simulink model "straperr"  (Simulink 7.9)
settings: Solver=ode23s  StartTime=0.0  StopTime=793  FixedStep=1  RelTol=1e-3
undefined symbols (not defined in the file or in its folder): D0, dcm2lat, dcm2lon, dcm2pitch, dcm2roll, dcm2yaw, getElem, plumbbobg, skew
libraries: simulink x2
settings Model: Creator=mcar  LastModifiedBy=1104070  ExtModeAutoUpdateStatusClock=off  BufferReuse=off
settings DataIOCC: ExternalInput=tu  LoadExternalInput=on  SaveFormat=StructureWithTime  SignalLoggingName=sigsOut
settings OptimizationCC: BlockReduction=off  BooleanDataType=off  OptimizeBlockIOStorage=off  BufferReuse=off  ExpressionFolding=off  LocalBlockOutputs=off
settings DebuggingCC: SaveWithParameterizedLinksMsg=none  SignalResolutionControl=TryResolveAllWithWarning  SolverPrmCheckMsg=none  MultiTaskDSMMsg=warning  MultiTaskCondExecSysMsg=none  StrictBusMsg=None
settings HardwareCC: TargetUnknown=on
settings RTWCC: IncludeERTFirstTime=on
settings GRTTargetCC: CombineOutputUpdateFcns=off  GRTInterface=on

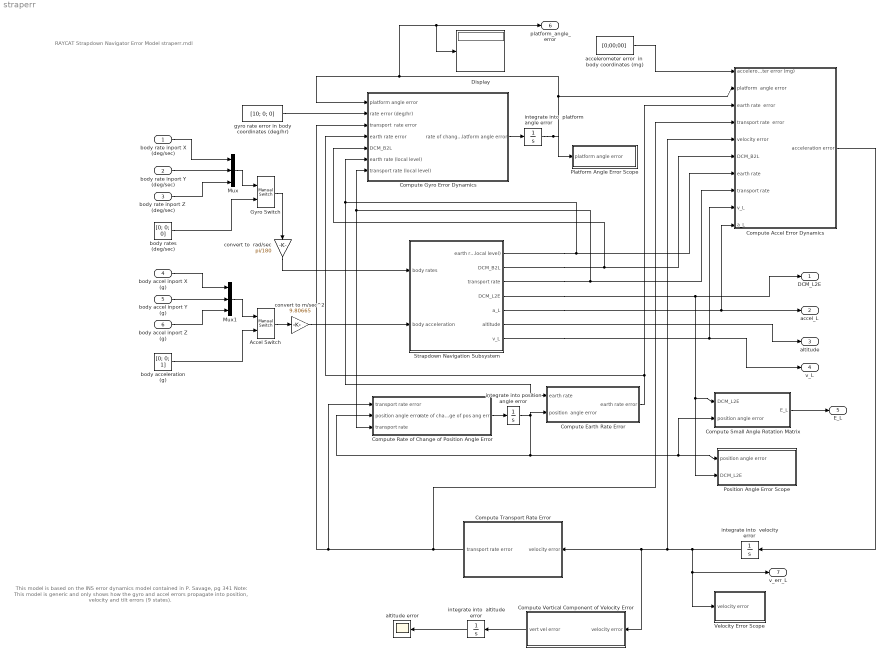
== system straperr ==
  note: RAYCAT Strapdown Navigator Error Model
      | straperr.mdl
  note: This model is based on the INS
      | error dynamics model contained in P. Savage, pg 341
      | Note:  This model is generic and only
      | shows how the gyro and accel errors propagate
      | into position, velocity and tilt errors (9 states).
  body rate inport X (deg/sec) : Inport
  body rate inport Y (deg/sec) : Inport  Port=2
  body rate inport Z  (deg/sec) : Inport  Port=3
  body accel inport X (g) : Inport  Port=4
  body accel inport Y (g) : Inport  Port=5
  body accel inport Z (g) : Inport  Port=6
  Accel Switch : simulink/Signal Routing/Manual Switch  sw=1  action=0  varsize=off
  Compute Accel Error Dynamics : Subsystem
  Compute Earth Rate Error : Subsystem
  Compute Gyro Error Dynamics : Subsystem
  Compute Rate of Change of Position Angle Error : Subsystem
  Compute Small Angle Rotation Matrix : Subsystem
  Compute Transport Rate Error : Subsystem
  Compute Vertical Component of Velocity Error : Subsystem
  Display : Display
  Gyro Switch : simulink/Signal Routing/Manual Switch  sw=1  action=0  varsize=off
  Mux : Mux  Inputs=3
  Mux1 : Mux  Inputs=3
  Platform Angle Error Scope : Subsystem
  Position Angle Error Scope : Subsystem
  Strapdown Navigation Subsystem : Subsystem  AncestorBlock=strapnavlib/Strapdown Navigation Subsystem
  Velocity Error Scope : Subsystem
  accelerometer error  in body coordinates (mg) : Constant  Value=[0;00;00]  VectorParams1D=off
  altitude error : Scope
      settings: YMin=-1  YMax=1
  body acceleration (g) : Constant  Value=[0; 0; 1]  VectorParams1D=off
  body rates (deg/sec) : Constant  Value="[0; 0;  0]"  VectorParams1D=off
  convert to  rad/sec : Gain  Gain=pi/180  SaturateOnIntegerOverflow=on  OutDataTypeStr=Inherit: Same as input  ParamDataTypeStr=Inherit: Same as input
  convert to m/sec^2 : Gain  Gain=9.80665  SaturateOnIntegerOverflow=on  OutDataTypeStr=Inherit: Same as input  ParamDataTypeStr=Inherit: Same as input
  gyro rate error in body coordinates (deg/hr) : Constant  Value=[10; 0; 0]  VectorParams1D=off
  integrate into position angle error : Integrator  InitialCondition=[0;0;0]
  integrate into  altitude error : Integrator  InitialCondition=[0;0;0]
  integrate into  platform angle error : Integrator  InitialCondition=[0;0;0]
  integrate into  velocity error : Integrator  InitialCondition=[0;0;0]
  DCM_L2E : Outport
  accel_L : Outport  Port=2
  altitude : Outport  Port=3
  v_L : Outport  Port=4
  E_L : Outport  Port=5
  platform_angle_error : Outport  Port=6
  v_err_L : Outport  Port=7
  wires:
  gyro rate error in body coordinates (deg/hr)/1 -> Compute Gyro Error Dynamics/2(rate error (deg/hr))
  Compute Gyro Error Dynamics/1(rate of change of platform angle error) -> integrate into  platform angle error/1
  integrate into  platform angle error/1 -> Platform Angle Error Scope/1(platform angle error), Compute Accel Error Dynamics/2(platform  angle error), Compute Gyro Error Dynamics/1(platform angle error), platform_angle_error/1, Display/1
  Compute Accel Error Dynamics/1(acceleration error) -> integrate into  velocity error/1
  integrate into  velocity error/1 -> Compute Transport Rate Error/1(velocity error), Compute Vertical Component of Velocity Error/1(velocity error), Compute Accel Error Dynamics/5(velocity error), Velocity Error Scope/1(velocity error), v_err_L/1
  Compute Vertical Component of Velocity Error/1(vert vel error) -> integrate into  altitude error/1
  accelerometer error  in body coordinates (mg)/1 -> Compute Accel Error Dynamics/1(accelerometer error (mg))
  Compute Transport Rate Error/1(transport rate error) -> Compute Gyro Error Dynamics/3(transport  rate error), Compute Rate of Change of Position Angle Error/1(transport rate error), Compute Accel Error Dynamics/4(transport rate  error)
  Compute Rate of Change of Position Angle Error/1(rate of change of pos ang err) -> integrate into position angle error/1
  integrate into  altitude error/1 -> altitude error/1
  Compute Earth Rate Error/1(earth rate error) -> Compute Gyro Error Dynamics/4(earth rate error), Compute Accel Error Dynamics/3(earth rate  error)
  Strapdown Navigation Subsystem/2(DCM_B2L) -> Compute Gyro Error Dynamics/5(DCM_B2L), Compute Accel Error Dynamics/6(DCM_B2L)
  Strapdown Navigation Subsystem/1(earth rate (local level)) -> Compute Gyro Error Dynamics/6(earth rate (local level)), Compute Earth Rate Error/1(earth rate), Compute Accel Error Dynamics/7(earth rate)
  Strapdown Navigation Subsystem/3(transport rate) -> Compute Accel Error Dynamics/8(transport rate), Compute Gyro Error Dynamics/7(transport rate (local level)), Compute Rate of Change of Position Angle Error/3(transport rate)
  integrate into position angle error/1 -> Compute Rate of Change of Position Angle Error/2(position angle error), Position Angle Error Scope/1(position angle error), Compute Small Angle Rotation Matrix/2(position angle error), Compute Earth Rate Error/2(position  angle error)
  Strapdown Navigation Subsystem/7(v_L) -> Compute Accel Error Dynamics/9(v_L), v_L/1
  Strapdown Navigation Subsystem/6(altitude) -> altitude/1
  Strapdown Navigation Subsystem/5(a_L) -> accel_L/1, Compute Accel Error Dynamics/10(a_L)
  Strapdown Navigation Subsystem/4(DCM_L2E) -> DCM_L2E/1, Position Angle Error Scope/2(DCM_L2E), Compute Small Angle Rotation Matrix/1(DCM_L2E)
  convert to  rad/sec/1 -> Strapdown Navigation Subsystem/1(body rates)
  convert to m/sec^2/1 -> Strapdown Navigation Subsystem/2(body acceleration)
  Compute Small Angle Rotation Matrix/1(E_L) -> E_L/1
  body rates (deg/sec)/1 -> Gyro Switch/2
  Gyro Switch/1 -> convert to  rad/sec/1
  Accel Switch/1 -> convert to m/sec^2/1
  body acceleration (g)/1 -> Accel Switch/2
  body rate inport Z  (deg/sec)/1 -> Mux/3
  body rate inport Y (deg/sec)/1 -> Mux/2
  body rate inport X (deg/sec)/1 -> Mux/1
  Mux/1 -> Gyro Switch/1
  body accel inport X (g)/1 -> Mux1/1
  body accel inport Y (g)/1 -> Mux1/2
  body accel inport Z (g)/1 -> Mux1/3
  Mux1/1 -> Accel Switch/1

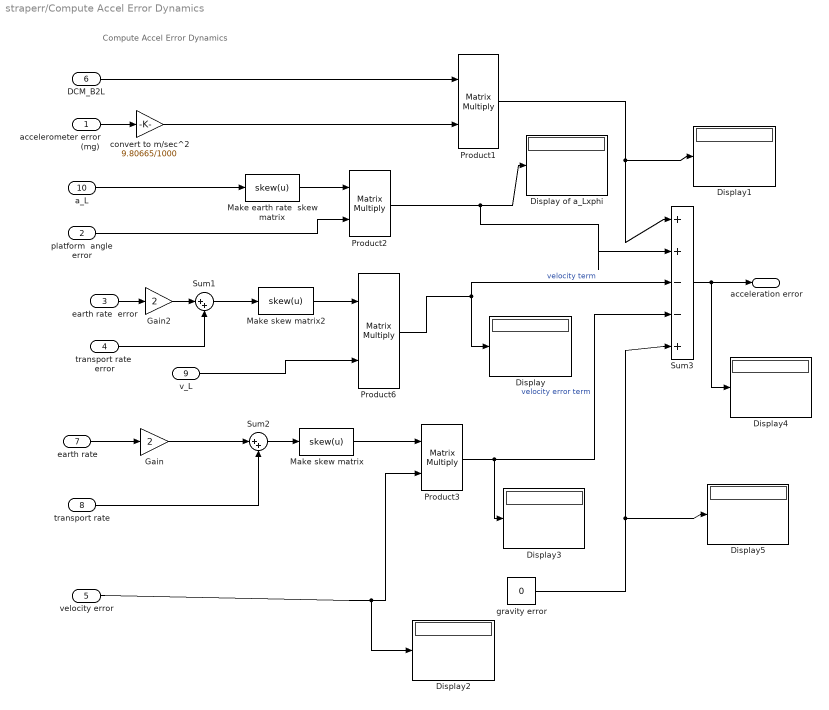
== system straperr/Compute Accel Error Dynamics ==
  note: Compute Accel Error Dynamics
  accelerometer error (mg) : Inport
  platform  angle error : Inport  Port=2
  earth rate  error : Inport  Port=3
  transport rate  error : Inport  Port=4
  velocity error : Inport  Port=5
  DCM_B2L : Inport  Port=6
  earth rate : Inport  Port=7
  transport rate : Inport  Port=8
  v_L : Inport  Port=9
  a_L : Inport  Port=10
  Display{,1..5} (6 alike) : Display
  Display of a_Lxphi : Display
  Gain : Gain  Gain=2  SaturateOnIntegerOverflow=on  OutDataTypeStr=Inherit: Same as input  ParamDataTypeStr=Inherit: Same as input
  Gain2 : Gain  Gain=2  SaturateOnIntegerOverflow=on  OutDataTypeStr=Inherit: Same as input  ParamDataTypeStr=Inherit: Same as input
  Make earth rate  skew matrix : MATLABFcn  MATLABFcn=skew(u)  Output1D=off
  Make skew matrix : MATLABFcn  MATLABFcn=skew(u)  Output1D=off
  Make skew matrix2 : MATLABFcn  MATLABFcn=skew(u)  Output1D=off
  Product{1..3,6} (4 alike) : Product  Multiplication=Matrix(*)  SaturateOnIntegerOverflow=on  InputSameDT=on  OutDataTypeStr=Inherit: Same as first input
  Sum1 : Sum  Inputs=|++  SaturateOnIntegerOverflow=on  InputSameDT=on  OutDataTypeStr=Inherit: Same as first input
  Sum2 : Sum  Inputs=|++  SaturateOnIntegerOverflow=on  InputSameDT=on  OutDataTypeStr=Inherit: Same as first input
  Sum3 : Sum  Inputs=|++--+  SaturateOnIntegerOverflow=on  InputSameDT=on  OutDataTypeStr=Inherit: Same as first input
  convert to m/sec^2 : Gain  Gain=9.80665/1000  SaturateOnIntegerOverflow=on  OutDataTypeStr=Inherit: Same as input  ParamDataTypeStr=Inherit: Same as input
  gravity error : Constant  Value=0
  acceleration error : Outport
  wires:
  accelerometer error (mg)/1 -> convert to m/sec^2/1
  Make earth rate  skew matrix/1 -> Product2/1
  platform  angle error/1 -> Product2/2
  Gain/1 -> Sum2/1
  Sum2/1 -> Make skew matrix/1
  Make skew matrix/1 -> Product3/1
  velocity error/1 -> Product3/2, Display2/1
  earth rate  error/1 -> Gain2/1
  Gain2/1 -> Sum1/1
  transport rate  error/1 -> Sum1/2
  Sum1/1 -> Make skew matrix2/1
  Sum3/1 -> acceleration error/1, Display4/1
  Product1/1 -> Sum3/1, Display1/1
  Product2/1 -> Sum3/2, Display of a_Lxphi/1
  gravity error/1 -> Sum3/5, Display5/1
  Product3/1 -> Sum3/4, Display3/1  "velocity error term"
  Product6/1 -> Sum3/3, Display/1  "velocity term"
  DCM_B2L/1 -> Product1/1
  earth rate/1 -> Gain/1
  transport rate/1 -> Sum2/2
  v_L/1 -> Product6/2
  convert to m/sec^2/1 -> Product1/2
  a_L/1 -> Make earth rate  skew matrix/1
  Make skew matrix2/1 -> Product6/1

== system straperr/Compute Earth Rate Error ==
  earth rate : Inport
  position  angle error : Inport  Port=2
  Gain : Gain  Gain=-1  SaturateOnIntegerOverflow=on  OutDataTypeStr=Inherit: Same as input  ParamDataTypeStr=Inherit: Same as input
  Make skew : MATLABFcn  MATLABFcn=skew(u)  Output1D=off
  Product : Product  Multiplication=Matrix(*)  SaturateOnIntegerOverflow=on  InputSameDT=on  OutDataTypeStr=Inherit: Same as first input
  earth rate error : Outport
  wires:
  position  angle error/1 -> Gain/1
  Gain/1 -> Make skew/1
  Make skew/1 -> Product/1
  earth rate/1 -> Product/2
  Product/1 -> earth rate error/1

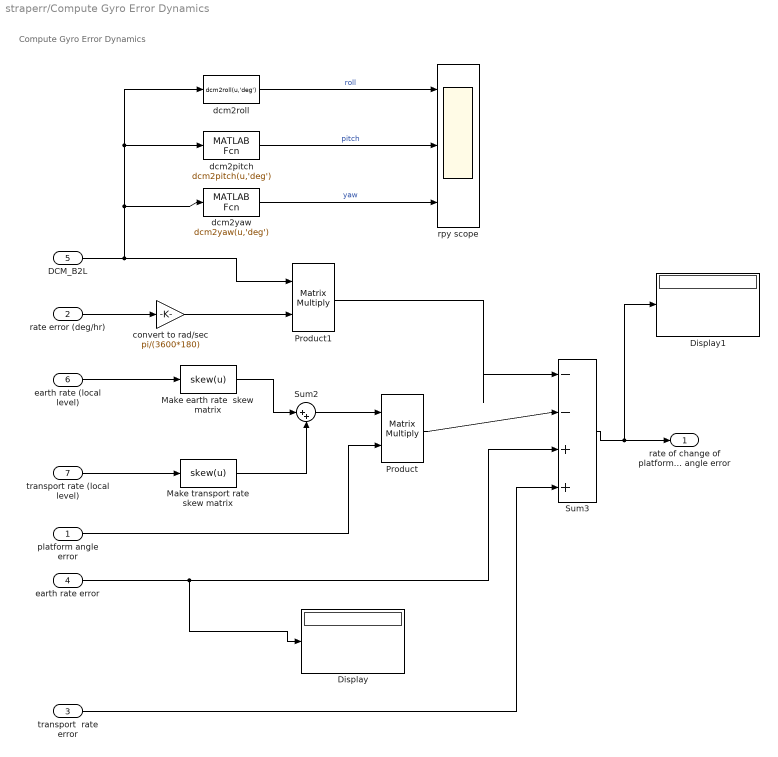
== system straperr/Compute Gyro Error Dynamics ==
  note: Compute Gyro Error Dynamics
  platform angle error : Inport
  rate error (deg/hr) : Inport  Port=2
  transport  rate error : Inport  Port=3
  earth rate error : Inport  Port=4
  DCM_B2L : Inport  Port=5
  earth rate (local level) : Inport  Port=6
  transport rate (local level) : Inport  Port=7
  Display : Display
  Display1 : Display
  Make earth rate  skew matrix : MATLABFcn  MATLABFcn=skew(u)  Output1D=off
  Make transport rate skew matrix : MATLABFcn  MATLABFcn=skew(u)  Output1D=off
  Product : Product  Multiplication=Matrix(*)  SaturateOnIntegerOverflow=on  InputSameDT=on  OutDataTypeStr=Inherit: Same as first input
  Product1 : Product  Multiplication=Matrix(*)  SaturateOnIntegerOverflow=on  InputSameDT=on  OutDataTypeStr=Inherit: Same as first input
  Sum2 : Sum  Inputs=|++  SaturateOnIntegerOverflow=on  InputSameDT=on  OutDataTypeStr=Inherit: Same as first input
  Sum3 : Sum  Inputs=|--++  SaturateOnIntegerOverflow=on  InputSameDT=on  OutDataTypeStr=Inherit: Same as first input
  convert to rad/sec : Gain  Gain=pi/(3600*180)  SaturateOnIntegerOverflow=on  OutDataTypeStr=Inherit: Same as input  ParamDataTypeStr=Inherit: Same as input
  dcm2pitch : MATLABFcn  MATLABFcn=dcm2pitch(u,'deg')  Output1D=off
  dcm2roll : MATLABFcn  MATLABFcn=dcm2roll(u,'deg')  Output1D=off
  dcm2yaw : MATLABFcn  MATLABFcn=dcm2yaw(u,'deg')  Output1D=off
  rpy scope : Scope  NumInputPorts=3
      settings: TimeRange=3600  YMin=-1~-1~0  YMax=1~1~20  SaveName=ScopeData2  MaxDataPoints=10000
  rate of change of platform angle error : Outport
  wires:
  Make transport rate skew matrix/1 -> Sum2/2
  Make earth rate  skew matrix/1 -> Sum2/1
  platform angle error/1 -> Product/2
  Sum2/1 -> Product/1
  rate error (deg/hr)/1 -> convert to rad/sec/1
  Product1/1 -> Sum3/1
  Sum3/1 -> rate of change of platform angle error/1, Display1/1
  transport  rate error/1 -> Sum3/4
  earth rate error/1 -> Sum3/3, Display/1
  DCM_B2L/1 -> Product1/1, dcm2yaw/1, dcm2pitch/1, dcm2roll/1
  earth rate (local level)/1 -> Make earth rate  skew matrix/1
  transport rate (local level)/1 -> Make transport rate skew matrix/1
  Product/1 -> Sum3/2
  dcm2roll/1 -> rpy scope/1  "roll"
  dcm2pitch/1 -> rpy scope/2  "pitch"
  dcm2yaw/1 -> rpy scope/3  "yaw"
  convert to rad/sec/1 -> Product1/2

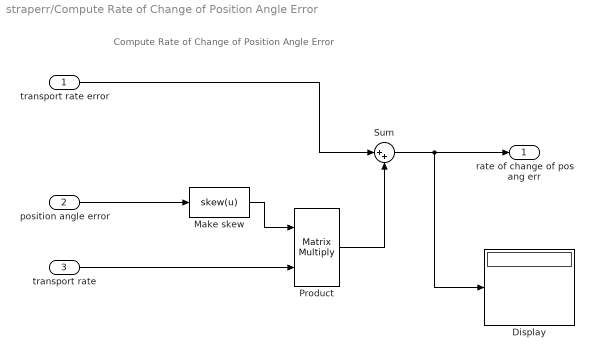
== system straperr/Compute Rate of Change of Position Angle Error ==
  note: Compute Rate of Change of Position Angle Error
  transport rate error : Inport
  position angle error : Inport  Port=2
  transport rate : Inport  Port=3
  Display : Display
  Make skew : MATLABFcn  MATLABFcn=skew(u)  Output1D=off
  Product : Product  Multiplication=Matrix(*)  SaturateOnIntegerOverflow=on  InputSameDT=on  OutDataTypeStr=Inherit: Same as first input
  Sum : Sum  Inputs=|++  SaturateOnIntegerOverflow=on  InputSameDT=on  OutDataTypeStr=Inherit: Same as first input
  rate of change of pos ang err : Outport
  wires:
  position angle error/1 -> Make skew/1
  Make skew/1 -> Product/1
  transport rate error/1 -> Sum/1
  Product/1 -> Sum/2
  Sum/1 -> rate of change of pos ang err/1, Display/1
  transport rate/1 -> Product/2

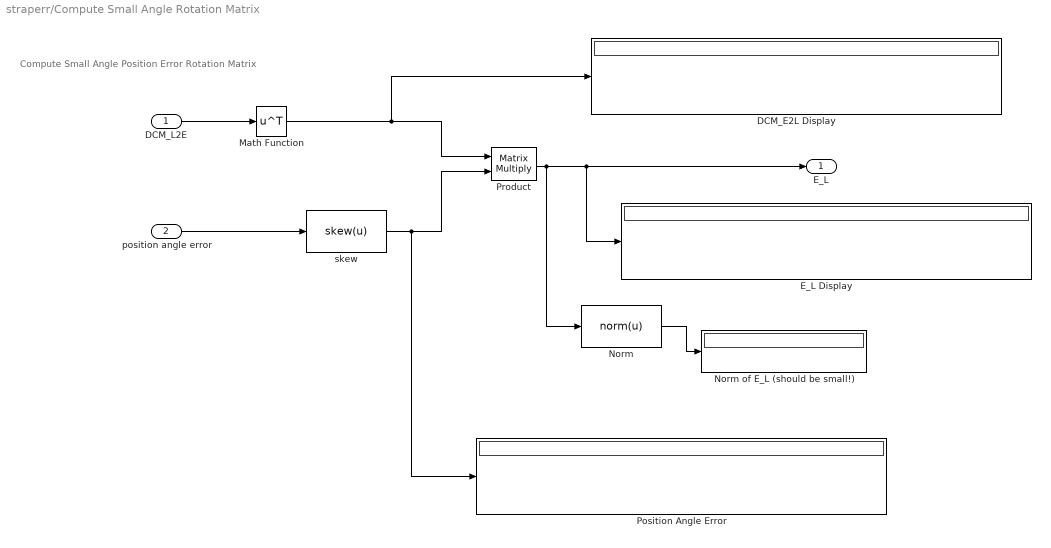
== system straperr/Compute Small Angle Rotation Matrix ==
  note: Compute Small Angle
      | Position Error
      | Rotation Matrix
  DCM_L2E : Inport
  position angle error : Inport  Port=2
  DCM_E2L Display : Display
  E_L Display : Display
  Math Function : Math  Operator=transpose  SaturateOnIntegerOverflow=on
  Norm : MATLABFcn  MATLABFcn=norm(u)  Output1D=off
  Norm of E_L (should be small!) : Display
  Position Angle Error : Display
  Product : Product  Multiplication=Matrix(*)  SaturateOnIntegerOverflow=on  InputSameDT=on  OutDataTypeStr=Inherit: Same as first input
  skew : MATLABFcn  MATLABFcn=skew(u)  Output1D=off
  E_L : Outport
  wires:
  DCM_L2E/1 -> Math Function/1
  Math Function/1 -> Product/1, DCM_E2L Display/1
  Product/1 -> E_L/1, E_L Display/1, Norm/1
  position angle error/1 -> skew/1
  skew/1 -> Product/2, Position Angle Error/1
  Norm/1 -> Norm of E_L (should be small!)/1

== system straperr/Compute Transport Rate Error ==
  velocity error : Inport
  1/R : Gain  Gain=1/6378137  SaturateOnIntegerOverflow=on  OutDataTypeStr=Inherit: Same as input  ParamDataTypeStr=Inherit: Same as input
  Constant1 : Constant  Value=[0 0 1]'  VectorParams1D=off
  Make skew : MATLABFcn  MATLABFcn=skew(u)  Output1D=off
  Product : Product  Multiplication=Matrix(*)  SaturateOnIntegerOverflow=on  InputSameDT=on  OutDataTypeStr=Inherit: Same as first input
  transport rate error : Outport
  wires:
  velocity error/1 -> Product/2
  Constant1/1 -> Make skew/1
  Product/1 -> transport rate error/1
  1/R/1 -> Product/1
  Make skew/1 -> 1/R/1

== system straperr/Compute Vertical Component of Velocity Error ==
  velocity error : Inport
  Dot Product : DotProduct  InputSameDT=on  OutDataTypeStr=Inherit: Inherit via internal rule
  unit vertical : Constant  Value=[0 0 1]'  VectorParams1D=off
  vert vel error : Outport
  wires:
  velocity error/1 -> Dot Product/2  "v_L"
  unit vertical/1 -> Dot Product/1
  Dot Product/1 -> vert vel error/1

== system straperr/Platform Angle Error Scope ==
  platform angle error : Inport
  Demux : Demux  Outputs=3
  Display of Platform Angle Error : Scope  NumInputPorts=3
      settings: TimeRange=10  YMin=-1.25538e+85~-2.69599e+67~-1  YMax=-0.422354~9e+83~1  SaveName=ScopeData5
  rad2deg : Gain  Gain=180/pi  SaturateOnIntegerOverflow=on  OutDataTypeStr=Inherit: Same as input  ParamDataTypeStr=Inherit: Same as input
  wires:
  platform angle error/1 -> rad2deg/1
  Demux/1 -> Display of Platform Angle Error/1
  Demux/2 -> Display of Platform Angle Error/2
  Demux/3 -> Display of Platform Angle Error/3
  rad2deg/1 -> Demux/1

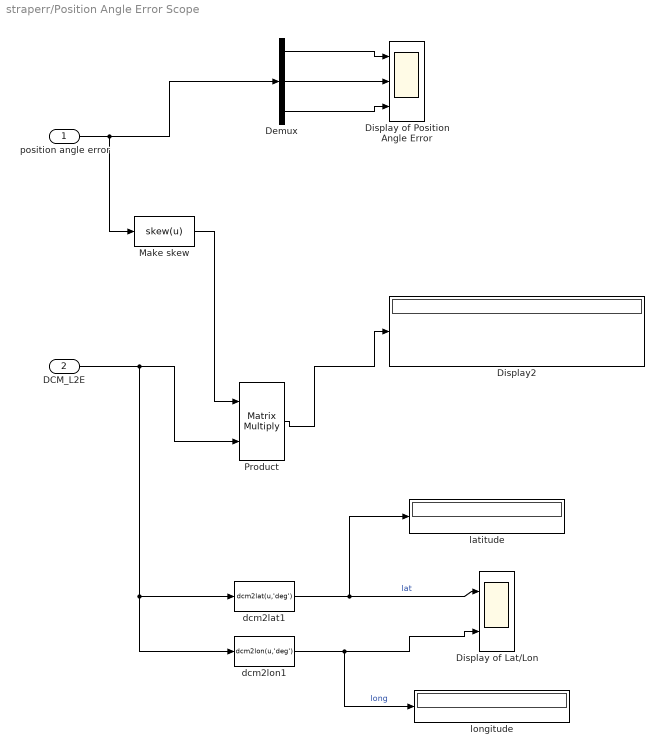
== system straperr/Position Angle Error Scope ==
  position angle error : Inport
  DCM_L2E : Inport  Port=2
  Demux : Demux  Outputs=3
  Display of Lat/Lon : Scope  NumInputPorts=2
      settings: YMin=-1~-1  YMax=1~1  SaveName=ScopeData10  MaxDataPoints=20000
  Display of Position Angle Error : Scope  NumInputPorts=3
      settings: YMin=-2.5e-09~0~-1  YMax=0~1.75e-12~1  SaveName=ScopeData5  MaxDataPoints=20000
  Display2 : Display
  Make skew : MATLABFcn  MATLABFcn=skew(u)  Output1D=off
  Product : Product  Multiplication=Matrix(*)  SaturateOnIntegerOverflow=on  InputSameDT=on  OutDataTypeStr=Inherit: Same as first input
  dcm2lat1 : MATLABFcn  MATLABFcn=dcm2lat(u,'deg')
  dcm2lon1 : MATLABFcn  MATLABFcn=dcm2lon(u,'deg')
  latitude : Display
  longitude : Display
  wires:
  Demux/3 -> Display of Position Angle Error/3
  Demux/2 -> Display of Position Angle Error/2
  Demux/1 -> Display of Position Angle Error/1
  position angle error/1 -> Demux/1, Make skew/1
  DCM_L2E/1 -> Product/2, dcm2lat1/1, dcm2lon1/1
  Make skew/1 -> Product/1
  Product/1 -> Display2/1
  dcm2lon1/1 -> longitude/1, Display of Lat/Lon/2  "long"
  dcm2lat1/1 -> latitude/1, Display of Lat/Lon/1  "lat"

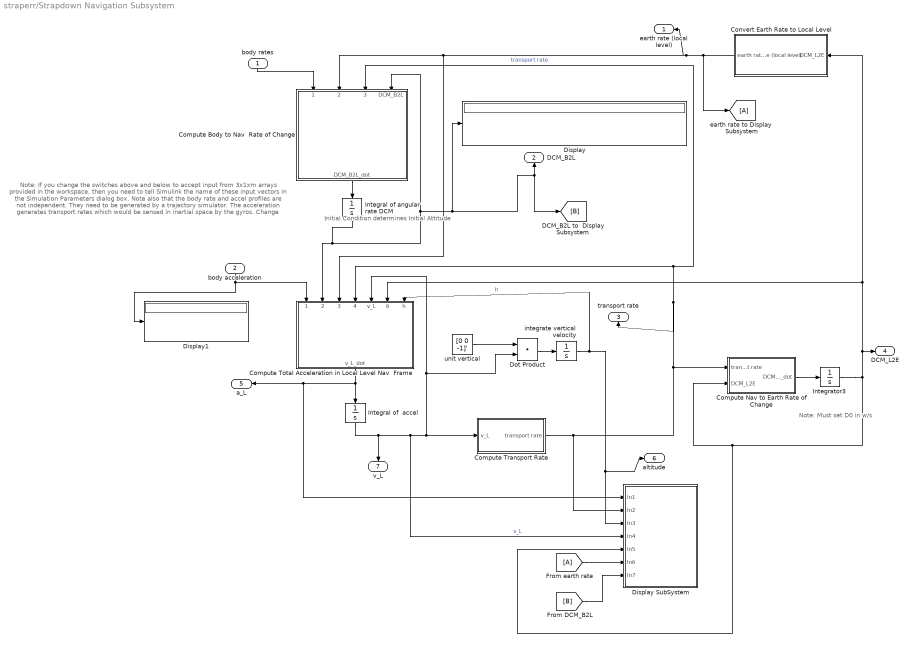
== system straperr/Strapdown Navigation Subsystem ==
  note: Note: If you change
      | the switches above and below
      | to accept input from 3x1xm
      | arrays provided in the workspace, then
      | you need to tell Simulink the name of these
      | input vectors in the Simulation Parameters
      | dialog box.
      | Note also that the body rate and accel
      | profiles are not independent.  They need
      | to be generated by a trajectory simulator.
      | The acceleration generates transport rates
      | which would be sensed in inertial space
      | by the gyros.
      | Change
  note: Initial
      | Condition
      | determines
      | Initial
      | Attitude
  note: Note:  Must set
      | D0 in w/s
  body rates : Inport
  body acceleration : Inport  Port=2
  Compute Body to Nav  Rate of Change : Subsystem
  Compute Nav to Earth Rate of Change : Subsystem
  Compute Total Acceleration in Local Level Nav  Frame : Subsystem
  Compute Transport Rate : Subsystem
  Convert Earth Rate to Local Level : Subsystem
  Display : Display
  Display SubSystem : Subsystem
  Display1 : Display
  Dot Product : DotProduct  InputSameDT=on  OutDataTypeStr=Inherit: Inherit via internal rule
  Integral of angular rate DCM : Integrator  InitialCondition=eye(3)
  Integral of  accel : Integrator  InitialCondition=[0 0 0]'
  Integrator3 : Integrator  InitialCondition=D0
  integrate vertical velocity : Integrator
  unit vertical : Constant  Value=[0 0 -1]'  VectorParams1D=off
  earth rate (local level) : Outport
  DCM_B2L : Outport  Port=2
  transport rate : Outport  Port=3
  DCM_L2E : Outport  Port=4
  a_L : Outport  Port=5
  altitude : Outport  Port=6
  v_L : Outport  Port=7
  wires:
  body acceleration/1 -> Compute Total Acceleration in Local Level Nav  Frame/1(accel_B), Display1/1
  body rates/1 -> Compute Body to Nav  Rate of Change/1(body rates)
  [B] -> Display SubSystem/7(In7)
  [A] -> Display SubSystem/6(In6)
  integrate vertical velocity/1 -> altitude/1, Display SubSystem/3(In3), Compute Total Acceleration in Local Level Nav  Frame/7(h)  "h"
  Convert Earth Rate to Local Level/1(earth rate (local level)) -> [A], earth rate (local level)/1, Compute Total Acceleration in Local Level Nav  Frame/3(earth rate), Compute Body to Nav  Rate of Change/2(earth rate)
  Integrator3/1 -> Display SubSystem/5(In5), Compute Nav to Earth Rate of Change/2(DCM_L2E), DCM_L2E/1, Convert Earth Rate to Local Level/1(DCM_L2E), Compute Total Acceleration in Local Level Nav  Frame/6(DCM_L2E)
  Compute Nav to Earth Rate of Change/1(DCM_L2E_dot) -> Integrator3/1
  Dot Product/1 -> integrate vertical velocity/1
  unit vertical/1 -> Dot Product/1
  Compute Transport Rate/1(transport rate) -> Display SubSystem/2(In2), transport rate/1, Compute Total Acceleration in Local Level Nav  Frame/4(transport rate), Compute Body to Nav  Rate of Change/3(transport rate), Compute Nav to Earth Rate of Change/1(transport rate)  "transport rate"
  Integral of  accel/1 -> v_L/1, Display SubSystem/4(In4), Compute Total Acceleration in Local Level Nav  Frame/5(v_L), Dot Product/2, Compute Transport Rate/1(v_L)  "v_L"
  Compute Total Acceleration in Local Level Nav  Frame/1(v_L_dot) -> a_L/1, Display SubSystem/1(In1), Integral of  accel/1
  Compute Body to Nav  Rate of Change/1(DCM_B2L_dot) -> Integral of angular rate DCM/1
  Integral of angular rate DCM/1 -> Compute Body to Nav  Rate of Change/4(DCM_B2L), DCM_B2L/1, [B], Display/1, Compute Total Acceleration in Local Level Nav  Frame/2(DCM_B2L)

== system straperr/Velocity Error Scope ==
  velocity error : Inport
  Demux : Demux  Outputs=3
  Display of Velocity Error : Scope  NumInputPorts=3
      settings: YMin=0~0~-0.05  YMax=350~20~0.03  SaveName=ScopeData5
  wires:
  velocity error/1 -> Demux/1
  Demux/1 -> Display of Velocity Error/1
  Demux/2 -> Display of Velocity Error/2
  Demux/3 -> Display of Velocity Error/3

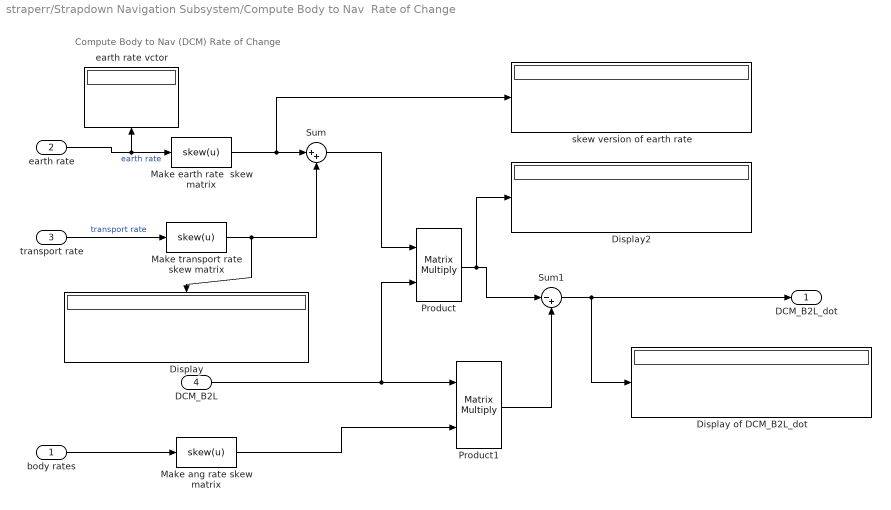
== system straperr/Strapdown Navigation Subsystem/Compute Body to Nav  Rate of Change ==
  note: Compute Body to Nav (DCM) Rate of Change
  body rates : Inport
  earth rate : Inport  Port=2
  transport rate : Inport  Port=3
  DCM_B2L : Inport  Port=4
  Display : Display
  Display of DCM_B2L_dot : Display
  Display2 : Display
  Make ang rate skew matrix : MATLABFcn  MATLABFcn=skew(u)  Output1D=off
  Make earth rate  skew matrix : MATLABFcn  MATLABFcn=skew(u)  Output1D=off
  Make transport rate skew matrix : MATLABFcn  MATLABFcn=skew(u)  Output1D=off
  Product : Product  Multiplication=Matrix(*)  SaturateOnIntegerOverflow=on  InputSameDT=on  OutDataTypeStr=Inherit: Same as first input
  Product1 : Product  Multiplication=Matrix(*)  SaturateOnIntegerOverflow=on  InputSameDT=on  OutDataTypeStr=Inherit: Same as first input
  Sum : Sum  Inputs=|++  SaturateOnIntegerOverflow=on  InputSameDT=on  OutDataTypeStr=Inherit: Same as first input
  Sum1 : Sum  Inputs=|-+  SaturateOnIntegerOverflow=on  InputSameDT=on  OutDataTypeStr=Inherit: Same as first input
  earth rate vctor : Display
  skew version of earth rate : Display
  DCM_B2L_dot : Outport
  wires:
  Sum1/1 -> DCM_B2L_dot/1, Display of DCM_B2L_dot/1
  Product1/1 -> Sum1/2
  Product/1 -> Sum1/1, Display2/1
  Make ang rate skew matrix/1 -> Product1/2
  Sum/1 -> Product/1
  DCM_B2L/1 -> Product1/1, Product/2
  Make earth rate  skew matrix/1 -> Sum/1, skew version of earth rate/1
  Make transport rate skew matrix/1 -> Sum/2, Display/1
  transport rate/1 -> Make transport rate skew matrix/1  "transport rate"
  earth rate/1 -> Make earth rate  skew matrix/1, earth rate vctor/1  "earth rate"
  body rates/1 -> Make ang rate skew matrix/1

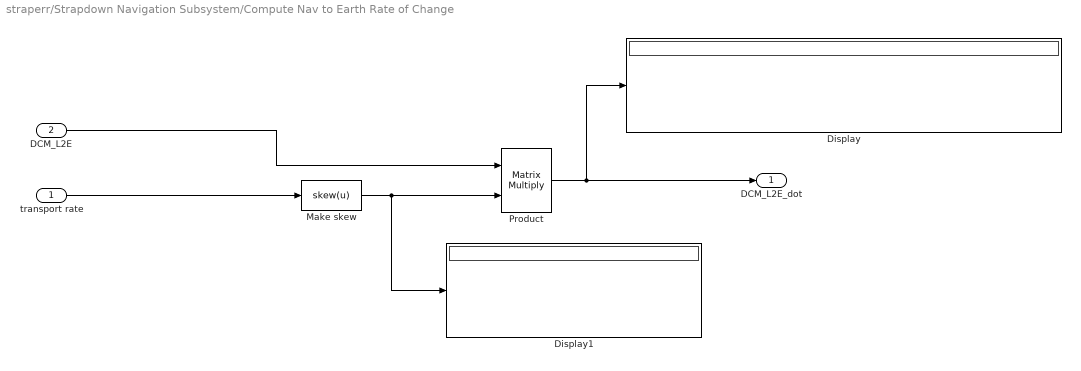
== system straperr/Strapdown Navigation Subsystem/Compute Nav to Earth Rate of Change ==
  transport rate : Inport
  DCM_L2E : Inport  Port=2
  Display : Display
  Display1 : Display
  Make skew : MATLABFcn  MATLABFcn=skew(u)  Output1D=off
  Product : Product  Multiplication=Matrix(*)  SaturateOnIntegerOverflow=on  InputSameDT=on  OutDataTypeStr=Inherit: Same as first input
  DCM_L2E_dot : Outport
  wires:
  DCM_L2E/1 -> Product/1
  transport rate/1 -> Make skew/1
  Make skew/1 -> Display1/1, Product/2
  Product/1 -> Display/1, DCM_L2E_dot/1

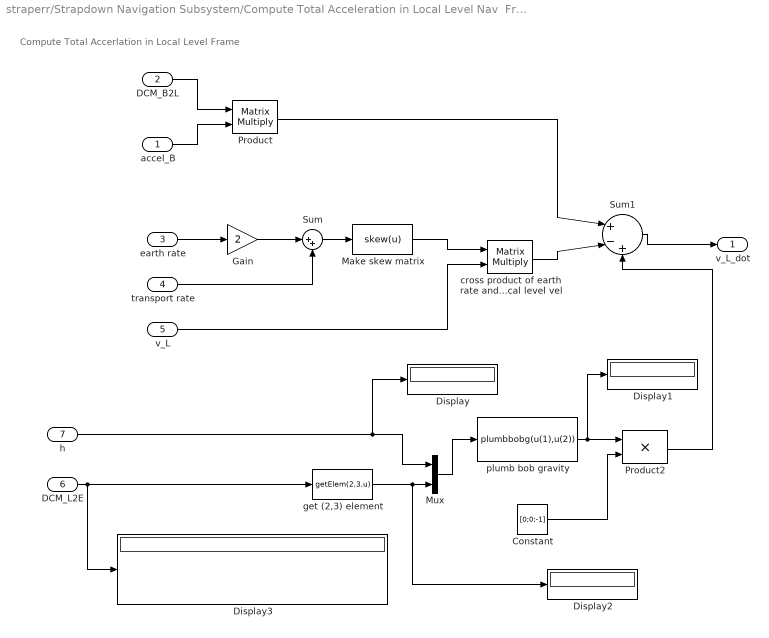
== system straperr/Strapdown Navigation Subsystem/Compute Total Acceleration in Local Level Nav  Frame ==
  note: Compute Total Accerlation in
      | Local Level Frame
  accel_B : Inport
  DCM_B2L : Inport  Port=2
  earth rate : Inport  Port=3
  transport rate : Inport  Port=4
  v_L : Inport  Port=5
  DCM_L2E : Inport  Port=6
  h : Inport  Port=7
  Constant : Constant  Value=[0;0;-1]  VectorParams1D=off
  Display{,1..3} (4 alike) : Display
  Gain : Gain  Gain=2  SaturateOnIntegerOverflow=on  OutDataTypeStr=Inherit: Same as input  ParamDataTypeStr=Inherit: Same as input
  Make skew matrix : MATLABFcn  MATLABFcn=skew(u)  Output1D=off
  Mux : Mux  Inputs=2
  Product : Product  Multiplication=Matrix(*)  SaturateOnIntegerOverflow=on  InputSameDT=on  OutDataTypeStr=Inherit: Same as first input
  Product2 : Product  SaturateOnIntegerOverflow=on  InputSameDT=on  OutDataTypeStr=Inherit: Same as first input
  Sum : Sum  Inputs=|++  SaturateOnIntegerOverflow=on  InputSameDT=on  OutDataTypeStr=Inherit: Same as first input
  Sum1 : Sum  Inputs=|+-+  SaturateOnIntegerOverflow=on  InputSameDT=on  OutDataTypeStr=Inherit: Same as first input
  cross product of earth rate and  transport rates  with local level vel : Product  Multiplication=Matrix(*)  SaturateOnIntegerOverflow=on  InputSameDT=on  OutDataTypeStr=Inherit: Same as first input
  get (2,3) element : MATLABFcn  MATLABFcn=getElem(2,3,u)  Output1D=off
  plumb bob gravity : MATLABFcn  MATLABFcn=plumbbobg(u(1),u(2))
  v_L_dot : Outport
  wires:
  Sum1/1 -> v_L_dot/1
  Product/1 -> Sum1/1
  cross product of earth rate and  transport rates  with local level vel/1 -> Sum1/2
  v_L/1 -> cross product of earth rate and  transport rates  with local level vel/2
  Make skew matrix/1 -> cross product of earth rate and  transport rates  with local level vel/1
  Sum/1 -> Make skew matrix/1
  transport rate/1 -> Sum/2
  Gain/1 -> Sum/1
  earth rate/1 -> Gain/1
  accel_B/1 -> Product/2
  DCM_B2L/1 -> Product/1
  DCM_L2E/1 -> get (2,3) element/1, Display3/1
  h/1 -> Mux/1, Display/1
  get (2,3) element/1 -> Mux/2, Display2/1
  Mux/1 -> plumb bob gravity/1
  Constant/1 -> Product2/2
  plumb bob gravity/1 -> Product2/1, Display1/1
  Product2/1 -> Sum1/3

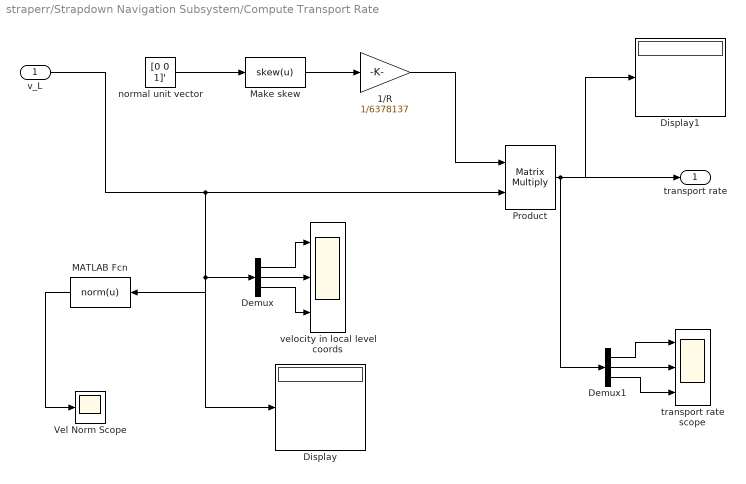
== system straperr/Strapdown Navigation Subsystem/Compute Transport Rate ==
  v_L : Inport
  1/R : Gain  Gain=1/6378137  SaturateOnIntegerOverflow=on  OutDataTypeStr=Inherit: Same as input  ParamDataTypeStr=Inherit: Same as input
  Demux : Demux  Outputs=3
  Demux1 : Demux  Outputs=3
  Display : Display
  Display1 : Display
  MATLAB Fcn : MATLABFcn  MATLABFcn=norm(u)
  Make skew : MATLABFcn  MATLABFcn=skew(u)  Output1D=off
  Product : Product  Multiplication=Matrix(*)  SaturateOnIntegerOverflow=on  InputSameDT=on  OutDataTypeStr=Inherit: Same as first input
  Vel Norm Scope : Scope
      settings: YMin=587.5  YMax=630  SaveName=ScopeData7
  normal unit vector : Constant  Value=[0 0 1]'  VectorParams1D=off
  transport rate scope : Scope  NumInputPorts=3
      settings: YMin=5.5e-007~1.8e-007~-1  YMax=6.7e-007~2.15e-007~1  SaveName=ScopeData3
  velocity in local level coords : Scope  NumInputPorts=3
      settings: YMin=-100000~-2.5e+006~-2.5e+006  YMax=700000~250000~2.5e+006  SaveName=ScopeData4
  transport rate : Outport
  wires:
  Make skew/1 -> 1/R/1
  1/R/1 -> Product/1
  Product/1 -> Display1/1, transport rate/1, Demux1/1
  normal unit vector/1 -> Make skew/1
  v_L/1 -> Product/2, Display/1, Demux/1, MATLAB Fcn/1
  Demux/1 -> velocity in local level coords/1
  Demux/2 -> velocity in local level coords/2
  Demux/3 -> velocity in local level coords/3
  Demux1/1 -> transport rate scope/1
  Demux1/2 -> transport rate scope/2
  Demux1/3 -> transport rate scope/3
  MATLAB Fcn/1 -> Vel Norm Scope/1

== system straperr/Strapdown Navigation Subsystem/Convert Earth Rate to Local Level ==
  DCM_L2E : Inport
  Earth Rate : Constant  Value=[0,0,7.292115167e-5]'  VectorParams1D=off
  Product : Product  Multiplication=Matrix(*)  SaturateOnIntegerOverflow=on  InputSameDT=on  OutDataTypeStr=Inherit: Same as first input
  transpose : MATLABFcn  MATLABFcn=u'  Output1D=off
  earth rate (local level) : Outport
  wires:
  Earth Rate/1 -> Product/2
  DCM_L2E/1 -> transpose/1
  Product/1 -> earth rate (local level)/1
  transpose/1 -> Product/1

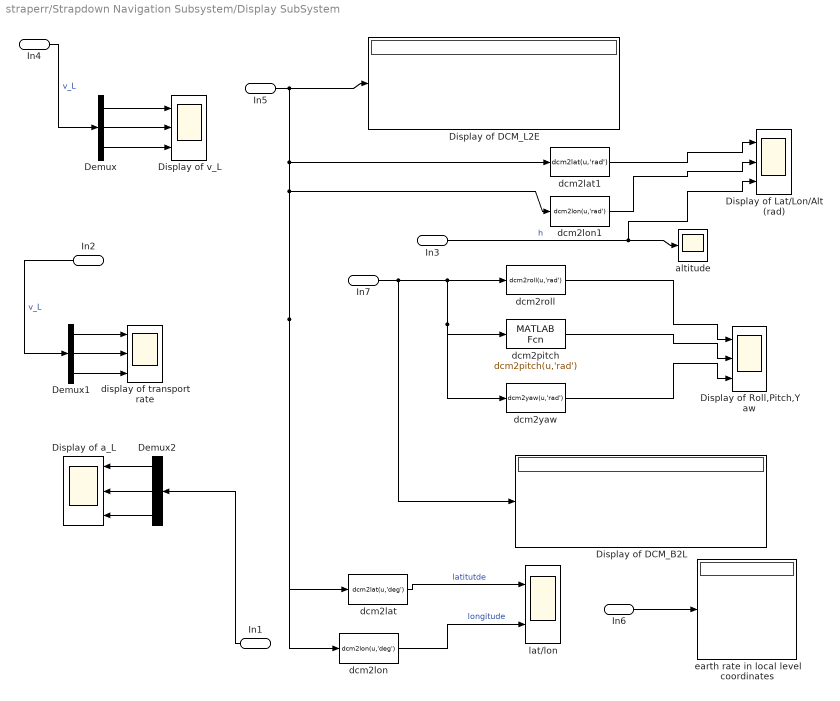
== system straperr/Strapdown Navigation Subsystem/Display SubSystem ==
  In1 : Inport
  In2 : Inport  Port=2
  In3 : Inport  Port=3
  In4 : Inport  Port=4
  In5 : Inport  Port=5
  In6 : Inport  Port=6
  In7 : Inport  Port=7
  Demux : Demux  Outputs=3
  Demux1 : Demux  Outputs=3
  Demux2 : Demux  Outputs=3
  Display of DCM_B2L : Display
  Display of DCM_L2E : Display
  Display of Lat/Lon/Alt (rad) : Scope  NumInputPorts=3
      settings: YMin=0~-0.13~0  YMax=0.04~0~3.5e+006  SaveName=ScopeData8
  Display of Roll,Pitch,Yaw : Scope  NumInputPorts=3
      settings: YMin=-0.1~0~-2.5e-009  YMax=0.1~0.2~1.5e-008  SaveName=ScopeData9
  Display of a_L : Scope  NumInputPorts=3
      settings: YMin=-5~-5~-5  YMax=5~5~5  SaveName=ScopeData2
  Display of v_L : Scope  NumInputPorts=3
      settings: YMin=-450~-100~-400  YMax=50~900~400  SaveName=ScopeData4
  altitude : Scope
      settings: TimeRange=1  YMin=-0.5  YMax=0
  dcm2lat : MATLABFcn  MATLABFcn=dcm2lat(u,'deg')
  dcm2lat1 : MATLABFcn  MATLABFcn=dcm2lat(u,'rad')
  dcm2lon : MATLABFcn  MATLABFcn=dcm2lon(u,'deg')
  dcm2lon1 : MATLABFcn  MATLABFcn=dcm2lon(u,'rad')
  dcm2pitch : MATLABFcn  MATLABFcn=dcm2pitch(u,'rad')
  dcm2roll : MATLABFcn  MATLABFcn=dcm2roll(u,'rad')
  dcm2yaw : MATLABFcn  MATLABFcn=dcm2yaw(u,'rad')
  display of transport rate : Scope  NumInputPorts=3
      settings: YMin=-5~-5~-5  YMax=5~5~5  SaveName=ScopeData3
  earth rate in local level coordinates : Display
  lat/lon : Scope  NumInputPorts=2
      settings: YMin=-5~-5  YMax=5~5
  wires:
  Demux2/3 -> Display of a_L/3
  Demux2/2 -> Display of a_L/2
  Demux2/1 -> Display of a_L/1
  In1/1 -> Demux2/1
  In3/1 -> altitude/1, Display of Lat/Lon/Alt (rad)/3  "h"
  In6/1 -> earth rate in local level coordinates/1
  In7/1 -> Display of DCM_B2L/1, dcm2roll/1, dcm2pitch/1, dcm2yaw/1
  In5/1 -> Display of DCM_L2E/1, dcm2lat1/1, dcm2lon/1, dcm2lat/1, dcm2lon1/1
  dcm2lon/1 -> lat/lon/2  "longitude"
  dcm2lat/1 -> lat/lon/1  "latitutde"
  Demux/3 -> Display of v_L/3
  Demux/2 -> Display of v_L/2
  Demux/1 -> Display of v_L/1
  In4/1 -> Demux/1  "v_L"
  Demux1/3 -> display of transport rate/3
  Demux1/2 -> display of transport rate/2
  Demux1/1 -> display of transport rate/1
  In2/1 -> Demux1/1  "v_L"
  dcm2lon1/1 -> Display of Lat/Lon/Alt (rad)/2
  dcm2lat1/1 -> Display of Lat/Lon/Alt (rad)/1
  dcm2roll/1 -> Display of Roll,Pitch,Yaw/1
  dcm2pitch/1 -> Display of Roll,Pitch,Yaw/2
  dcm2yaw/1 -> Display of Roll,Pitch,Yaw/3
